simulink model "phi1_m2_vr001_k5_2"  (R2026a)
settings: Solver=VariableStepAuto  StopTime=24.0
libraries: deeplib x1
settings Model: Creator=ldy  LastModifiedBy=harry_31916
settings DataIOCC: OutputTimes=tspan

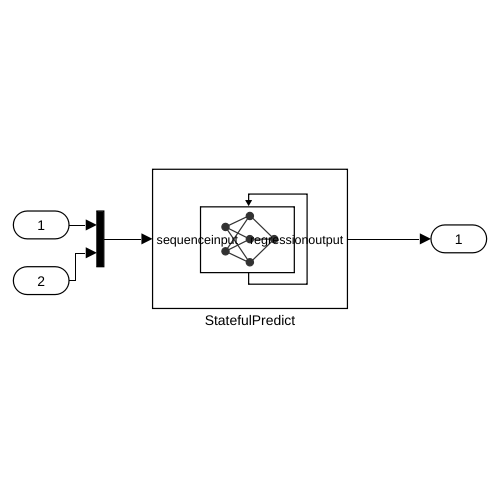
[thumbnail: Simulink's stored preview of the top-level diagram]
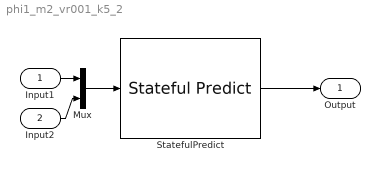
== system phi1_m2_vr001_k5_2 ==
  Input1 : Inport
  Input2 : Inport  Port=2
  Mux : Mux  Inputs=2
  StatefulPredict : deeplib/Stateful Predict  Network=Network from MAT-file  NetworkFunction=untitled  NetworkFilePath=phi1_m2_vr001_k5_2.mat  SimulateUsing=Auto mode  InputDataFormats={'',''}  SampleTime=1  ForceInterpretedSim=off  EnableDLNetwork=on  LastKnownNetworkFilePath=''  LastKnownNetworkTimeStamp=''
  Output : Outport
  wires:
  Input1/1 -> Mux/1
  Input2/1 -> Mux/2
  Mux/1 -> StatefulPredict/1
  StatefulPredict/1 -> Output/1
